simulink model "pmsm_foc_simulink"  (R2020b)
settings: Solver=ode4  StartTime=0.0  StopTime=3  FixedStep=1e-05  RelTol=1e-3
values from neighbouring files (symbols this model uses):
  fault = evalin('base', 'fault')    [run_simulink_simulation.m]
  motor = evalin('base', 'motor')    [run_simulink_mpc_simulation.m]
  profile = evalin('base', 'profile')    [run_simulink_mpc_simulation.m]    (also in run_simulink_simulation.m)
settings Model: Creator=arpankailashgupta  LastModifiedBy=arpankailashgupta
settings DataIOCC: SaveOutput=off

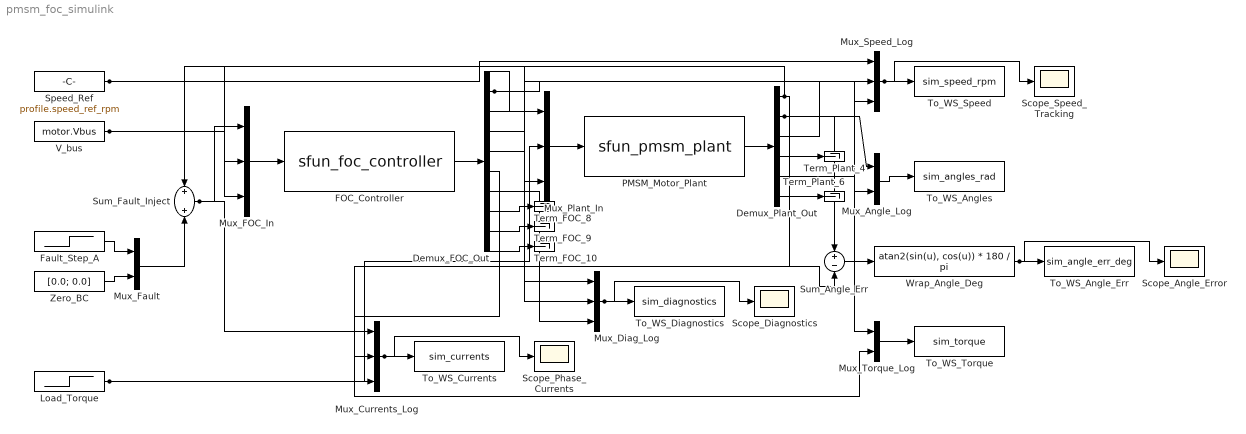
== system pmsm_foc_simulink ==
  Demux_FOC_Out : Demux  Outputs=[3, 1, 1, 1, 1, 3, 1, 2, 2, 2]
  Demux_Plant_Out : Demux  Outputs=[3, 1, 1, 1, 1, 2]
  FOC_Controller : S-Function  FunctionName=sfun_foc_controller  Parameters=MotorParamVec, CtrlParamVec, sim_cfg.Ts_ctrl  SFunctionDeploymentMode=off  EnableBusSupport=off
  Fault_Step_A : Step  Time=fault.onset_time  Before=0.0  After=fault.offset_val * fault.enable  SampleTime=0
  Load_Torque : Step  Time=profile.load_step_time  Before=0.0  After=profile.load_torque_Nm  SampleTime=0
  Mux_Angle_Log : Mux  Inputs=2
  Mux_Currents_Log : Mux  Inputs=3
  Mux_Diag_Log : Mux  Inputs=3
  Mux_FOC_In : Mux  Inputs=3
  Mux_Fault : Mux  Inputs=2
  Mux_Plant_In : Mux  Inputs=3
  Mux_Speed_Log : Mux  Inputs=3
  Mux_Torque_Log : Mux  Inputs=2
  PMSM_Motor_Plant : S-Function  FunctionName=sfun_pmsm_plant  Parameters=MotorParamVec, motor.Tcog  SFunctionDeploymentMode=off  EnableBusSupport=off
  Scope_Angle_Error : Scope
  Scope_Diagnostics : Scope
  Scope_Phase_Currents : Scope
  Scope_Speed_Tracking : Scope
  Speed_Ref : Constant  Value=profile.speed_ref_rpm
  Sum_Angle_Err : Sum  Inputs=+-
  Sum_Fault_Inject : Sum
  Term_FOC_10 : Terminator
  Term_FOC_8 : Terminator
  Term_FOC_9 : Terminator
  Term_Plant_4 : Terminator
  Term_Plant_6 : Terminator
  To_WS_Angle_Err : ToWorkspace  VariableName=sim_angle_err_deg  SampleTime=-1
  To_WS_Angles : ToWorkspace  VariableName=sim_angles_rad  SampleTime=-1
  To_WS_Currents : ToWorkspace  VariableName=sim_currents  SampleTime=-1
  To_WS_Diagnostics : ToWorkspace  VariableName=sim_diagnostics  SampleTime=-1
  To_WS_Speed : ToWorkspace  VariableName=sim_speed_rpm  SampleTime=-1
  To_WS_Torque : ToWorkspace  VariableName=sim_torque  SampleTime=-1
  V_bus : Constant  Value=motor.Vbus
  Wrap_Angle_Deg : Fcn  Expr=atan2(sin(u), cos(u)) * 180 / pi
  Zero_BC : Constant  Value=[0.0; 0.0]
  wires:
  Fault_Step_A/1 -> Mux_Fault/1
  Zero_BC/1 -> Mux_Fault/2
  Demux_Plant_Out/1 -> Sum_Fault_Inject/1, Mux_Currents_Log/3
  Mux_Fault/1 -> Sum_Fault_Inject/2
  Sum_Fault_Inject/1 -> Mux_FOC_In/1, Mux_Currents_Log/1
  V_bus/1 -> Mux_FOC_In/2, Mux_Plant_In/3
  Speed_Ref/1 -> Mux_FOC_In/3, Mux_Speed_Log/1
  Mux_FOC_In/1 -> FOC_Controller/1
  FOC_Controller/1 -> Demux_FOC_Out/1
  Demux_FOC_Out/1 -> Mux_Plant_In/1
  Load_Torque/1 -> Mux_Plant_In/2, Mux_Torque_Log/2
  Mux_Plant_In/1 -> PMSM_Motor_Plant/1
  PMSM_Motor_Plant/1 -> Demux_Plant_Out/1
  Demux_Plant_Out/3 -> Mux_Speed_Log/2
  Demux_FOC_Out/3 -> Mux_Speed_Log/3
  Mux_Speed_Log/1 -> To_WS_Speed/1, Scope_Speed_Tracking/1
  Demux_Plant_Out/2 -> Mux_Angle_Log/1, Sum_Angle_Err/1
  Demux_FOC_Out/2 -> Mux_Angle_Log/2, Sum_Angle_Err/2
  Mux_Angle_Log/1 -> To_WS_Angles/1
  Sum_Angle_Err/1 -> Wrap_Angle_Deg/1
  Wrap_Angle_Deg/1 -> To_WS_Angle_Err/1, Scope_Angle_Error/1
  Demux_FOC_Out/6 -> Mux_Currents_Log/2
  Mux_Currents_Log/1 -> To_WS_Currents/1, Scope_Phase_Currents/1
  Demux_FOC_Out/4 -> Mux_Diag_Log/1
  Demux_FOC_Out/5 -> Mux_Diag_Log/2
  Demux_FOC_Out/7 -> Mux_Diag_Log/3
  Mux_Diag_Log/1 -> To_WS_Diagnostics/1, Scope_Diagnostics/1
  Demux_Plant_Out/5 -> Mux_Torque_Log/1
  Mux_Torque_Log/1 -> To_WS_Torque/1
  Demux_FOC_Out/8 -> Term_FOC_8/1
  Demux_FOC_Out/9 -> Term_FOC_9/1
  Demux_FOC_Out/10 -> Term_FOC_10/1
  Demux_Plant_Out/4 -> Term_Plant_4/1
  Demux_Plant_Out/6 -> Term_Plant_6/1
